simulink model "motorDrivelineElectricalTRQControl"  (R2025b)
settings: Solver=VariableStepAuto  StartTime=0.0  StopTime=0.5  FixedStep=Ts  RelTol=1e-3  AbsTol=1e-3  EnableMultiTasking=on
PreLoadFcn:
  | motorDrivelineElectricalTRQControlParams;
undefined symbols (not defined in the file): elecTRQParams
libraries: nesl_utility x12, fl_lib x10, ee_lib x4, batteryecm_lib x1, eePmsmFieldOrientedControl x1
CloseFcn:
  | try,close(h1_PMSMDrive),end
  | clear h1_PMSMDrive
  | try,close(h2_PMSMDrive),end
  | clear h2_PMSMDrive
  | try,close(h3_PMSMDrive),end
  | clear h3_PMSMDrive
  | try,close(h4_PMSMDrive),end
  | clear h4_PMSMDrive
Description:
  | Three-Phase PMSM Drive
settings Model: Creator=The MathWorks, Inc.  LastModifiedBy=shachind
settings SolverCC: AutoScaleAbsTol=off  MaxConsecutiveMinStep=2  ZeroCrossAlgorithm=Adaptive  AlgebraicLoopSolver=TrustRegion  MaxZcPerStep=1.0
settings DataIOCC: LimitDataPoints=on  MaxDataPoints=690000  SaveFormat=Array  SignalLogging=off
settings OptimizationCC: ReuseModelBlockBuffer=off  LifeSpan=inf
settings DebuggingCC: MaxConsecutiveZCsMsg=none  IgnoredZcDiagnostic=none  UnconnectedInputMsg=warning  UnconnectedOutputMsg=warning  UnconnectedLineMsg=warning  AllowSymbolicDim=off  PregeneratedLibrarySubsystemCodeDiagnostic=none  SFUnexpectedBacktrackingDiag=warning  SFNoUnconditionalDefaultTransitionDiag=warning  SFExecutionAtInitializationDiag=none  ArithmeticOperatorsInVariantConditions=warning
settings HardwareCC: ProdBitPerPointer=32.0  ProdBitPerSizeT=32.0  ProdBitPerPtrDiffT=32.0  ProdLargestAtomicFloat=None  ProdIntDivRoundTo=Undefined  ProdEndianess=Unspecified  ProdWordSize=32.0  ProdHWDeviceType=32-bit Generic
settings ModelReferenceCC: EnableRefExpFcnMdlSchedulingChecks=on  PropagateSignalLabelsOutOfModel=off
settings SFSimCC: SimUseLocalCustomCode=off
settings RTWCC: RTWUseLocalCustomCode=off  GPUComputeCapability=3.5  DLArmComputeVersion=19.05
settings CodeAppCC: StateflowObjectComments=on
settings GRTTargetCC: TargetLangStandard=C89/C90 (ANSI)
settings ConfigComp: CovMetricSettings=dw  CovSaveCumulativeToWorkspaceVar=on  CovSaveSingleToWorkspaceVar=on  CovExternalEMLEnable=off  CovSFcnEnable=off
settings SimscapeCC: SimscapeLogType=all  SimscapeLogName=simlogmotorDrivelineElectricalTRQControl  SimscapeLogLimitData=off  SimscapeLogDataHistory=690000.0

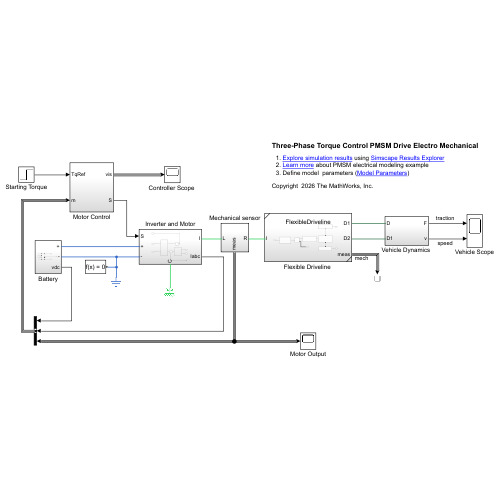
[thumbnail: Simulink's stored preview of the top-level diagram]
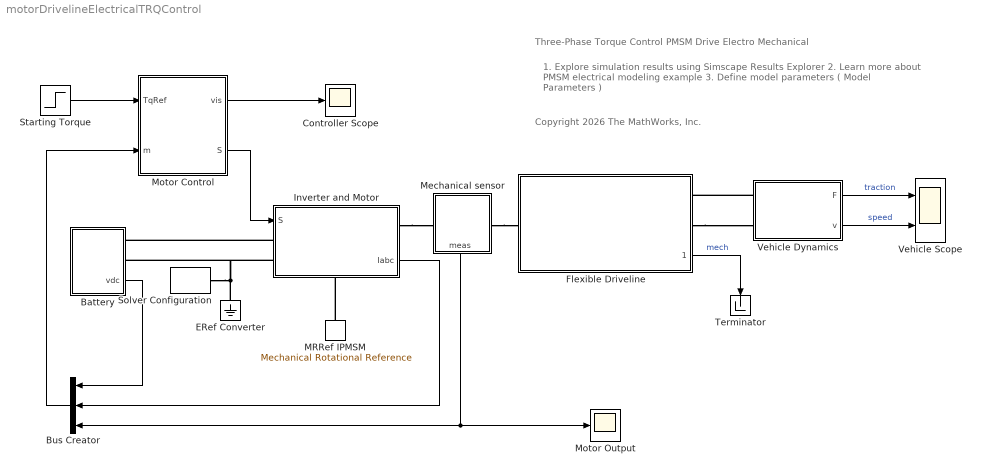
== system motorDrivelineElectricalTRQControl ==
  note: Three-Phase Torque Control PMSM Drive Electro Mechanical
  note: 1. Explore simulation results using Simscape Results Explorer
      | 2. Learn more about PMSM electrical modeling example
      | 3. Define model parameters ( Model Parameters )
  note: Copyright 2026 The MathWorks, Inc.
  Battery : Subsystem
      settings: PortSchema="{\"entries\":[{\"content\":{\"sides\":[{\"content\":{},\"type\":\"ConnectorPlacement.EquallySpacedRectSide\",\"uuid\":\"3e4692f5-9bd7-4a52-b9b4-dbfde3041e1b\"},{\"content\":{\"connectorIds\":[\"RConn1\",\"RConn2\",\"Out1\"],\"side\":\"RIGHT\"},\"type\":\"ConnectorPlacement.EquallySpacedRectSide\",\"uuid\":\"34170655-efd1-4725-b892-0490a88cd6b3\"},{\"content\":{\"side\":\"TOP\"},\"type\":\"ConnectorPlacement.EquallySpacedRectSide\",\"uuid\":\"051e7fe0-e37a-4958-8dcf-c73d0495e662\"},{\"content\":{\"side\":\"BOTTOM\"},\"type\":\"ConnectorPlacement.EquallySpacedRectSide\",\"uuid\":\"b1fc2594-e254-4206-a57f-073d724655f5\"}]},\"type\":\"ConnectorPlacement.EquallySpacedConnector\",\"uuid\":\"32af2e3c-f8f5-43b3-81bc-9b6fee978ebc\"}],\"packageUris\":[\"http://schema.mathworks.com/mf0/Connector/R2020b\"],\"version\":\"1.0\"}"
  Bus Creator : BusCreator  Inputs=3
  "Controller Scope " : Scope
      settings: ActiveDisplayYMinimum=-362.43334059575272  ActiveDisplayYMaximum=223.49886029038308
  ERef Converter : fl_lib/Electrical/Electrical Elements/Electrical Reference
  "Flexible Driveline " : Subsystem  ReferencedSubsystem=FlexibleDriveline
      settings: PortSchema="{\"entries\":[{\"content\":{\"sides\":[{\"content\":{\"connectorIds\":[\"LConn1\"]},\"type\":\"ConnectorPlacement.EquallySpacedRectSide\",\"uuid\":\"b641ef45-b70e-4196-8c46-ca8cab1c313e\"},{\"content\":{\"connectorIds\":[\"RConn1\",\"RConn2\",\"Out1\"],\"side\":\"RIGHT\"},\"type\":\"ConnectorPlacement.EquallySpacedRectSide\",\"uuid\":\"8a51df86-71ec-48ae-9cae-5a3f671581d5\"},{\"content\":{\"side\":\"TOP\"},\"type\":\"ConnectorPlacement.EquallySpacedRectSide\",\"uuid\":\"1e4e883b-852e-4889-9310-df4ba72c2f7b\"}]},\"type\":\"ConnectorPlacement.EquallySpacedConnector\",\"uuid\":\"d094a044-8f93-4a08-a2c2-1a95b6407718\"}],\"packageUris\":[\"http://schema.mathworks.com/mf0/Connector/R2020b\"],\"version\":\"1.0\"}"
  Inverter and Motor : Subsystem
      settings: PortSchema="{\"entries\":[{\"content\":{\"sides\":[{\"content\":{\"connectorIds\":[\"In1\",\"LConn1\",\"LConn2\"]},\"type\":\"ConnectorPlacement.EquallySpacedRectSide\",\"uuid\":\"79886a42-20e0-415e-bc70-e8f3f934141c\"},{\"content\":{\"connectorIds\":[\"RConn1\",\"Out1\"],\"side\":\"RIGHT\"},\"type\":\"ConnectorPlacement.EquallySpacedRectSide\",\"uuid\":\"24b2e8ac-3a57-4634-be65-eb2e006efc4c\"},{\"content\":{\"side\":\"TOP\"},\"type\":\"ConnectorPlacement.EquallySpacedRectSide\",\"uuid\":\"fad38467-7104-4348-9d8d-90e314d27ae8\"},{\"content\":{\"connectorIds\":[\"RConn2\"],\"side\":\"BOTTOM\"},\"type\":\"ConnectorPlacement.EquallySpacedRectSide\",\"uuid\":\"f364d779-702d-4da4-a90d-a3d412e5412e\"}]},\"type\":\"ConnectorPlacement.EquallySpacedConnector\",\"uuid\":\"c4c0e35c-7ac9-412b-ab3f-384c1c56da6e\"}],\"packageUris\":[\"http://schema.mathworks.com/mf0/Connector/R2020b\"],\"version\":\"1.0\"}"
  MRRef IPMSM : fl_lib/Mechanical/Rotational Elements/Mechanical Rotational Reference
  Mechanical sensor : Subsystem
      settings: PortSchema="{\"entries\":[{\"content\":{\"sides\":[{\"content\":{\"connectorIds\":[\"LConn1\"]},\"type\":\"ConnectorPlacement.EquallySpacedRectSide\",\"uuid\":\"9d0b7eaf-5dbc-4711-a9f9-5254d5ad2438\"},{\"content\":{\"connectorIds\":[\"RConn1\"],\"side\":\"RIGHT\"},\"type\":\"ConnectorPlacement.EquallySpacedRectSide\",\"uuid\":\"1084bd7e-accf-404d-815d-6b48331d5fd1\"},{\"content\":{\"side\":\"TOP\"},\"type\":\"ConnectorPlacement.EquallySpacedRectSide\",\"uuid\":\"4e1c109f-5704-45c2-8a88-7bde344122da\"},{\"content\":{\"connectorIds\":[\"Out1\"],\"side\":\"BOTTOM\"},\"type\":\"ConnectorPlacement.EquallySpacedRectSide\",\"uuid\":\"dec56fa8-46a5-4b4d-8685-27108f0f957c\"}]},\"type\":\"ConnectorPlacement.EquallySpacedConnector\",\"uuid\":\"e6b98985-8de9-437e-9e9a-976cda41402d\"}],\"packageUris\":[\"http://schema.mathworks.com/mf0/Connector/R2020b\"],\"version\":\"1.0\"}"
  Motor Control : Subsystem
  Motor Output : Scope
      settings: ActiveDisplayYMinimum=-152.33940612292497  ActiveDisplayYMaximum=237.58310712785936  DataLoggingVariableName=ScopeData2
  Solver Configuration : nesl_utility/Solver Configuration  PhysicalDomain=network_engine_domain  SubClassName=solver  LeftPortType=input  RightPortType=generic  Tones=[]  Harmonics=[]  SimulateNoise=off  Profile=off  UseLocalSampling=off  EnableSwitchedLinearOptims=on  FrequencyDomain=off  UseCCode=off  RelTol=0.001  AbsTol=0.001  MinStep=1e-09  ToWorkspace=off  RevertToSquareIcSolve=off  NumHomotopyIterations=100  PhasorMode=off  PhasorModeNumHarmonics=1  ConsistencySolver=NEWTON_XTOL_AFTER_FTOL  IndexReductionMethod=DerivativeReplacement  DoDC=off  ResidualTolerance=1e-09  ConsistencyTolSource=GLOBAL  ConsistencyAbsTol=0.001  ConsistencyRelTol=0.001  ConsistencyTolFactor=0.001  UseLocalSolver=on  LocalSolverChoice=NE_BACKWARD_EULER_ADVANCER  ResolveIndetEquations=on  FunctionEvalNumThread=1  LocalSolverSampleTime=5e-5  DoFixedCost=off  MaxNonlinIter=3  MaxModeIter=2  ComputeImpulses=off  ImpulseIterations=2  LinearAlgebra=auto  LinearAlgebraNumThread=0  EquationFormulation=NE_TIME_EF  DelaysMemoryBudget=1024  AutomaticFiltering=on  FilteringTimeConstant=0.001  PartitionStorageMethod=AS_NEEDED  PartitionMemoryBudget=1024  PartitionMethod=ROBUST  MultibodyUseLocalSolver=off  MultibodyLocalSolverChoice=ODE1  MultibodyLocalSolverSampleTime=0.001
  Starting Torque : Step  Time=0.01  After=50  SampleTime=0
  Terminator : Terminator
  "Vehicle Dynamics " : Subsystem
  Vehicle Scope : Scope  NumInputPorts=2
      settings: ActiveDisplayYMinimum=-534.32238927144817  ActiveDisplayYMaximum=4808.9015034430349
  wires:
  "Vehicle Dynamics "/1(F) -> Vehicle Scope/1  "traction"
  "Vehicle Dynamics "/2(v) -> Vehicle Scope/2  "speed"
  Bus Creator/1 -> Motor Control/2(m)
  Starting Torque/1 -> Motor Control/1(TqRef)
  Battery/1(vdc) -> Bus Creator/1
  Motor Control/2(S) -> Inverter and Motor/1(S)
  Inverter and Motor/1(Iabc) -> Bus Creator/2
  Mechanical sensor/1(meas) -> Motor Output/1, Bus Creator/3
  "Flexible Driveline "/1 -> Terminator/1  "mech"
  Motor Control/1(vis) -> "Controller Scope "/1
  connections:
  "Vehicle Dynamics "/LConn1 -- "Flexible Driveline "/RConn1
  "Flexible Driveline "/RConn2 -- "Vehicle Dynamics "/LConn2
  Solver Configuration/RConn1 -- ERef Converter/LConn1 -- Inverter and Motor/LConn2 -- Battery/RConn2
  Inverter and Motor/LConn1 -- Battery/RConn1
  MRRef IPMSM/LConn1 -- Inverter and Motor/RConn2
  Inverter and Motor/RConn1 -- Mechanical sensor/RConn1
  Mechanical sensor/LConn1 -- "Flexible Driveline "/LConn1

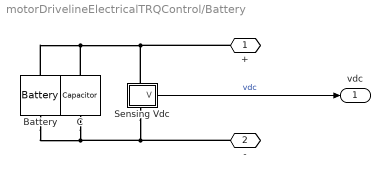
== system motorDrivelineElectricalTRQControl/Battery ==
  Battery : batteryecm_lib/Battery  Vnom=450 V  prm_dir=1  R1_dis=2 Ohm  R1_ch=2 Ohm  R1=0.001 Ohm  prm_AH=1  AH=300 hr*A  V1=V1 V  AH1=100 hr*A  prm_R2=1  R2=2000 Ohm  Tmeas=298.15 K  charge_measurement_port=simscape.enum.battery.enable.no  prm_dyn=1  Rp1=0.005 Ohm  tau1=30 s  Rp2=0.005 Ohm  tau2=30 s  Rp3=0.005 Ohm  tau3=30 s  Rp4=0.005 Ohm  tau4=30 s  Rp5=0.005 Ohm  tau5=30 s  prm_fade=1  N_fade=100  AH_fade=45 hr*A  R1_fade=2.02 Ohm  R1_ch_fade=2.02 Ohm  V1_fade=10.35 V  prm_age=1  prm_age_OCV=1  OCV_age=0.9  SOC_age=60  Tmeas_age=298.15 K  delta_time_age_vec=[0] d  temperature_age_vec=[273] K  OCV_scaling_age=2.2134e6  OCV_offset_age=1.632e6  temp_exp_age=0.515833569 V  t_exp_age=0.75  Vnom_T2=12 V  R1_T2=2.2 Ohm  R1_T2_dis=2.2 Ohm  R1_T2_ch=2.2 Ohm  V1_T2=11.4 V  R2_T2=2200 Ohm  Rp1_T2=0.005 Ohm  tau1_T2=30 s  Rp2_T2=0.005 Ohm  tau2_T2=30 s  Rp3_T2=0.005 Ohm  tau3_T2=30 s  Rp4_T2=0.005 Ohm  tau4_T2=30 s  Rp5_T2=0.005 Ohm  tau5_T2=30 s  Tmeas2=273.15 K  thermal_port=simscape.enum.thermaleffects.omit  thermal_mass=30000 J/K  i_specify=off  i_priority=None  i=0 A  i_nominal_specify=off  i_nominal_value=1  i_nominal_unit=A  v_specify=off  v_priority=None  v=0 V  v_nominal_specify=off  v_nominal_value=1  v_nominal_unit=V  charge_specify=on  charge_priority=High  charge=elecTRQParams.battery.ah0 hr*A  charge_nominal_specify=off  charge_nominal_value=1  charge_nominal_unit=A*hr  num_cycles_specify=off  num_cycles_priority=High  num_cycles=0  num_cycles_nominal_specify=off  num_cycles_nominal_value=1  num_cycles_nominal_unit=1  temperature_specify=off  temperature_priority=High  temperature=298.15 K  temperature_nominal_specify=off  temperature_nominal_value=1  temperature_nominal_unit=K
  C : fl_lib/Electrical/Electrical Elements/Capacitor  c=elecTRQParams.battery.cdc F  r=1e-6 Ohm  g=0 1/Ohm  i_specify=off  i_priority=None  i=0 A  i_nominal_specify=off  i_nominal_value=1  i_nominal_unit=A  v_specify=off  v_priority=None  v=0 V  v_nominal_specify=off  v_nominal_value=1  v_nominal_unit=V  vc_specify=on  vc_priority=None  vc=elecTRQParams.battery.vnom V  vc_nominal_specify=off  vc_nominal_value=1  vc_nominal_unit=V
  Sensing Vdc : Subsystem
      settings: PortSchema="{\"entries\":[{\"content\":{\"sides\":[{\"content\":{\"connectorIds\":[\"LConn1\"]},\"type\":\"ConnectorPlacement.EquallySpacedRectSide\",\"uuid\":\"bc3757cc-4537-444e-89af-7b7d8c8c1fa7\"},{\"content\":{\"connectorIds\":[\"RConn1\"],\"side\":\"RIGHT\"},\"type\":\"ConnectorPlacement.EquallySpacedRectSide\",\"uuid\":\"908bf4c4-26f6-4d8a-bcf8-68236027f5f8\"},{\"content\":{\"side\":\"TOP\"},\"type\":\"ConnectorPlacement.EquallySpacedRectSide\",\"uuid\":\"33f228db-ba47-4718-96dc-a72de309ae8c\"},{\"content\":{\"connectorIds\":[\"Out1\"],\"side\":\"BOTTOM\"},\"type\":\"ConnectorPlacement.EquallySpacedRectSide\",\"uuid\":\"d9b66c7e-0954-4c47-8bcc-77bf13ff573c\"}]},\"type\":\"ConnectorPlacement.EquallySpacedConnector\",\"uuid\":\"345f3578-0572-4e64-b2f3-84728129a12d\"}],\"packageUris\":[\"http://schema.mathworks.com/mf0/Connector/R2020b\"],\"version\":\"1.0\"}"
  + : PMIOPort  Side=Right
  - : PMIOPort  Port=2  Side=Right
  vdc : Outport
  wires:
  Sensing Vdc/1(V) -> vdc/1  "vdc"
  connections:
  C/LConn1 -- +/RConn1 -- Sensing Vdc/LConn1 -- Battery/LConn1
  -/RConn1 -- Battery/RConn1 -- C/RConn1 -- Sensing Vdc/RConn1

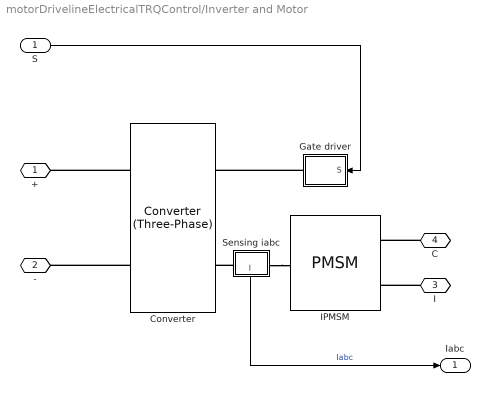
== system motorDrivelineElectricalTRQControl/Inverter and Motor ==
  S : Inport
  Converter : ee_lib/Semiconductors & Converters/Converters/Converter (Three-Phase)  port_option=ee.enum.threePhasePort.composite  fidelity_option=ee.enum.converters.fidelity.detailed  device_type=ee.enum.converters.switchingdevice.ideal  showThermalPort=false  K=0  Vth=0.5 V  Vgt=1 V  Vgt_off=-1 V  Ih=1 A  Vf=0.8 V  Ron=0.001 Ohm  Rds=0.001 Ohm  Goff=1e-5 1/Ohm  Eon_scalar=22.86e-3 J  Eoff_scalar=17.14e-3 J  Eoff_natural_commutation=10e-3 J  Voff=300 V  Iout_scalar=600 A  onCurrentMeasDelay=0 s  useCurrentFromPreviousCycle=false  useVoltageFromPreviousCycle=false  diode_param=ee.enum.converters.protectiondiode.nodynamics  diode_Vf=0.8 V  diode_Ron=0.001 Ohm  diode_Goff=1e-5 1/Ohm  diode_C=50 nF  diode_iRM=-235 A  diode_iF=300 A  diode_idot=-50 A/us  diode_trr_param=1  diode_trr_factor=3  diode_trr=15 us  diode_Qrr=1.5e+3 s*uA  diode_rec_loss_model=ee.enum.diode.reverseRecoveryModel.fixed  diode_ErecVal=0 J  diode_scaleWithIandV=false  diode_ErecMat=zeros(2, 3) J  diode_TjrecVec=[298.15, 398.15] K  diode_IfrecVec=[.1, 1, 10] A  diode_IrecVal=10 A  diode_VrecVal=10 V  diode_tFilter=1 / 1000 / 100 s  thermal_network_parameterization=ee.enum.thermalNetworkTopology.external  Rth=[.08, .5] K/W  Rth_Cauer=[.08, .1, .5] K/W  Rth_Foster=[.08, .14, .22, .16] K/W  thermal_mass_parameterization=ee.enum.thermalNetwork.timeconstant  thermal_mass=[.01, .5] J/K  thermal_mass_Cauer=[.01, .1, .5] J/K  thermal_mass_Foster=[.001, .005, .05, .5] J/K  thermal_time_constant=[.001, .2] s  thermal_time_constant_Cauer=[.001, .1, .2] s  thermal_time_constant_Foster=[7e-05, .0007, .01, .08] s  thermal_mass_initial_temperatures=[25, 25] degC  thermal_mass_initial_temperatures_Cauer=[25, 25, 25] degC  junction_thermal_mass=0.01 J/K  Tvec_initial_Foster=[25, 25, 25, 25] degC  snubber_type=0  Cs=1e-7 F  Rs=0.1 Ohm  Vce_loss=[0, 150, 300] V
  Gate driver : Subsystem
  IPMSM : ee_lib/Electromechanical/Permanent Magnet/PMSM  port_option=ee.enum.threePhasePort.composite  winding_type=ee.enum.statorconnection.wye  machine_param=ee.enum.pmsm.parameterization.constant  nPolePairs=elecTRQParams.motor.p  pmflux_param=ee.enum.pmflux.fluxlinkage  pm_flux_linkage=elecTRQParams.motor.psim Wb  torque_constant=0.18 N*m/A  back_emf_constant=0.18 V/(rad/s)  stator_param=ee.enum.statorparam.LdLqL0  Ld=elecTRQParams.motor.ld H  Lq=elecTRQParams.motor.lq H  idVec=[-200, 0, 200] A  iqVec=[-200, 0, 200] A  LdMatrix=0.0002 * ones(3, 3) H  LqMatrix=0.0002 * ones(3, 3) H  PmMatrix=0.1 * ones(3, 3) Wb  ktMatrix=0.18 * ones(3, 3) N*m/A  keMatrix=0.18 * ones(3, 3) V/(rad/s)  L0=elecTRQParams.motor.l0 H  Ls=0.0002 H  Lm=0.00002 H  Ms=0.00002 H  Rs=elecTRQParams.motor.rs Ohm  zero_sequence=ee.enum.park.zerosequence.exclude  axes_param=ee.enum.rotorangle.qaxis  loss_param=ee.enum.ironloss.none  losses_oc=[0, 0, 0] W  losses_sc=[0, 0, 0] W  f_losses=60 Hz  Isc_losses=95 A  J=0.01 kg*m^2  lam=0.1 N*m/(rad/s)  i_d_specify=off  i_d_priority=None  i_d=0 A  i_d_nominal_specify=off  i_d_nominal_value=1  i_d_nominal_unit=A  i_q_specify=off  i_q_priority=None  i_q=0 A  i_q_nominal_specify=off  i_q_nominal_value=1  i_q_nominal_unit=A  torque_specify=off  torque_priority=None  torque=0 N*m  torque_nominal_specify=off  torque_nominal_value=1  torque_nominal_unit=N*m  angular_velocity_specify=on  angular_velocity_priority=None  angular_velocity=0 rad/s  angular_velocity_nominal_specify=off  angular_velocity_nominal_value=1  angular_velocity_nominal_unit=rpm  angular_position_specify=on  angular_position_priority=High  angular_position=0 rad  angular_position_nominal_specify=off  angular_position_nominal_value=1  angular_position_nominal_unit=deg  alpha=3.93e-3 1/K  alpha_flux=-0.001 1/K  Tmeas=298.15 K  stator_thermal_mass=100 J/K  rotor_thermal_mass=200 J/K  Rm_percent_rotor=90  Rd_percent_rotor=30  temperatureA_specify=off  temperatureA_priority=High  temperatureA=25 degC  temperatureA_nominal_specify=off  temperatureA_nominal_value=1  temperatureA_nominal_unit=degC  temperatureB_specify=off  temperatureB_priority=High  temperatureB=25 degC  temperatureB_nominal_specify=off  temperatureB_nominal_value=1  temperatureB_nominal_unit=degC  temperatureC_specify=off  temperatureC_priority=High  temperatureC=25 degC  temperatureC_nominal_specify=off  temperatureC_nominal_value=1  temperatureC_nominal_unit=degC  temperatureR_specify=off  temperatureR_priority=High  temperatureR=25 degC  temperatureR_nominal_specify=off  temperatureR_nominal_value=1  temperatureR_nominal_unit=degC
      settings: InternalSimscapePortConfiguration="{\"Bottom\":[],\"Left\":[{\"id\":\"N\",\"label\":\"~\",\"type\":\"foundation.electrical.three_phase\"}],\"Right\":[{\"id\":\"R\",\"label\":\"R\",\"type\":\"foundation.mechanical.rotational.rotational\"},{\"id\":\"C\",\"label\":\"C\",\"type\":\"foundation.mechanical.rotational.rotational\"}],\"Top\":[]}"
  Sensing iabc : Subsystem
      settings: PortSchema="{\"entries\":[{\"content\":{\"sides\":[{\"content\":{\"connectorIds\":[\"LConn1\"]},\"type\":\"ConnectorPlacement.EquallySpacedRectSide\",\"uuid\":\"bc3757cc-4537-444e-89af-7b7d8c8c1fa7\"},{\"content\":{\"connectorIds\":[\"RConn1\"],\"side\":\"RIGHT\"},\"type\":\"ConnectorPlacement.EquallySpacedRectSide\",\"uuid\":\"908bf4c4-26f6-4d8a-bcf8-68236027f5f8\"},{\"content\":{\"connectorIds\":[],\"side\":\"TOP\"},\"type\":\"ConnectorPlacement.EquallySpacedRectSide\",\"uuid\":\"33f228db-ba47-4718-96dc-a72de309ae8c\"},{\"content\":{\"connectorIds\":[\"Out1\"],\"side\":\"BOTTOM\"},\"type\":\"ConnectorPlacement.EquallySpacedRectSide\",\"uuid\":\"3b1d40a5-3c80-431c-8111-df754e0c502b\"}]},\"type\":\"ConnectorPlacement.EquallySpacedConnector\",\"uuid\":\"345f3578-0572-4e64-b2f3-84728129a12d\"}],\"packageUris\":[\"http://schema.mathworks.com/mf0/Connector/R2020b\"],\"version\":\"1.0\"}"
  + : PMIOPort  Side=Left
  - : PMIOPort  Port=2  Side=Left
  I : PMIOPort  Port=3  Side=Right
  C : PMIOPort  Port=4  Side=Right
  Iabc : Outport
  wires:
  Sensing iabc/1(I) -> Iabc/1  "Iabc"
  S/1 -> Gate driver/1(S)
  connections:
  Sensing iabc/RConn1 -- IPMSM/LConn1
  C/RConn1 -- IPMSM/RConn2
  Converter/RConn2 -- -/RConn1
  Sensing iabc/LConn1 -- Converter/LConn2
  Gate driver/RConn1 -- Converter/LConn1
  Converter/RConn1 -- +/RConn1
  I/RConn1 -- IPMSM/RConn1

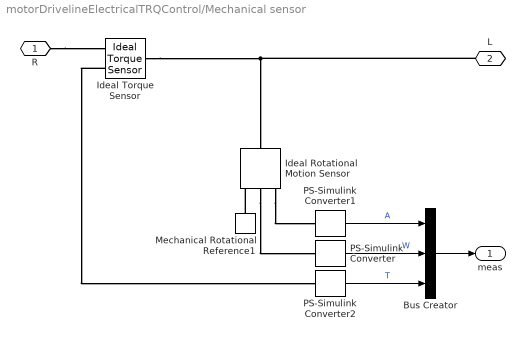
== system motorDrivelineElectricalTRQControl/Mechanical sensor ==
  Bus Creator : BusCreator  Inputs=3
  Ideal Rotational Motion Sensor : fl_lib/Mechanical/Mechanical Sensors/Ideal Rotational Motion Sensor  reference=foundation.enum.MeasurementReference.difference  acceleration_port=false  velocity_port=true  position_port=true  wrap_angle=simscape.enum.onoff.off  offset=0 deg
  Ideal Torque Sensor : fl_lib/Mechanical/Mechanical Sensors/Ideal Torque Sensor
  Mechanical Rotational Reference1 : fl_lib/Mechanical/Rotational Elements/Mechanical Rotational Reference
  PS-Simulink Converter : nesl_utility/PS-Simulink Converter  PhysicalDomain=network_engine_domain  SubClassName=ps_output  LeftPortType=input  RightPortType=output  PseudoPeriodic=off  Frequencies=[]  VectorFormat=1-D array  Unit=rad/s  AffineConversion=off
  PS-Simulink Converter1 : nesl_utility/PS-Simulink Converter  PhysicalDomain=network_engine_domain  SubClassName=ps_output  LeftPortType=input  RightPortType=output  PseudoPeriodic=off  Frequencies=[]  VectorFormat=1-D array  Unit=rad  AffineConversion=off
  PS-Simulink Converter2 : nesl_utility/PS-Simulink Converter  PhysicalDomain=network_engine_domain  SubClassName=ps_output  LeftPortType=input  RightPortType=output  PseudoPeriodic=off  Frequencies=[]  VectorFormat=1-D array  Unit=N*m  AffineConversion=off
  R : PMIOPort  Side=Left
  L : PMIOPort  Port=2  Side=Right
  meas : Outport  VectorParamsAs1DForOutWhenUnconnected=off
  wires:
  Bus Creator/1 -> meas/1
  PS-Simulink Converter1/1 -> Bus Creator/1  "A"
  PS-Simulink Converter/1 -> Bus Creator/2  "W"
  PS-Simulink Converter2/1 -> Bus Creator/3  "T"
  connections:
  L/RConn1 -- Ideal Torque Sensor/LConn1 -- Ideal Rotational Motion Sensor/LConn1
  Ideal Rotational Motion Sensor/RConn2 -- PS-Simulink Converter/LConn1
  Ideal Rotational Motion Sensor/RConn3 -- PS-Simulink Converter1/LConn1
  Mechanical Rotational Reference1/LConn1 -- Ideal Rotational Motion Sensor/RConn1
  Ideal Torque Sensor/RConn2 -- PS-Simulink Converter2/LConn1
  R/RConn1 -- Ideal Torque Sensor/RConn1

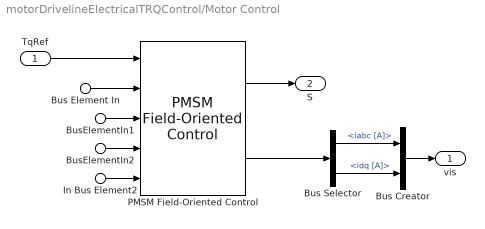
== system motorDrivelineElectricalTRQControl/Motor Control ==
  TqRef : Inport
  Bus Element In : Inport  Port=2  PortName=m  Element=Iabc
  In Bus Element2 : Inport  Port=2  PortName=m  Element=vdc
  BusElementIn1 : Inport  Port=2  PortName=m  Element=signal3.W
  BusElementIn2 : Inport  Port=2  PortName=m  Element=signal3.A
  Bus Creator : BusCreator  Inputs=2
  Bus Selector : BusSelector  OutputSignals=iabc [A],idq [A]
  PMSM Field-Oriented Control : eePmsmFieldOrientedControl/PMSM Field-Oriented Control  winding_type=Wye-wound  CtrlMode=Torque control  Vnom=elecTRQParams.battery.vnom  Pmax=28902.6524  Tmax=elecTRQParams.motor.tmax  p=elecTRQParams.motor.p  Vdc_on=100  Ts=elecTRQParams.control.ts  Tsc=elecTRQParams.control.tsc  CtrlType=PI control  Kp_w=1  Ki_w=1  Kv_w=1  Kaw_w=1  RefType=Zero d-axis control  rpmVec=[0, 3000]  TqVec=[-100, 0, 100]  VdcVec=[300, 350]  PWMMode=SVM: space vector modulation  ModFactor=1  idMatrix=zeros(2,3,2)  iqMatrix=zeros(2,3,2)  psim=elecTRQParams.motor.psim  Ld=0.00024  Lq=0.00029  Rs=0.01  AxisAlignment=Q-axis  Kp_id=elecTRQParams.piId.kp  Ki_id=elecTRQParams.piId.ki  Kaw_id=1  Kp_iq=elecTRQParams.piIq.kp  Ki_iq=elecTRQParams.piIq.ki  Kaw_iq=1  AxisPrio=Q-axis  ActZC=off  ActFF=on  ParamTypeFF=Constant parameters  LdFF=elecTRQParams.motor.ld  LqFF=elecTRQParams.motor.lq  psimFF=elecTRQParams.motor.psim  idVect=[-200, 0, 200]  iqVect=[-200, 0, 200]  LdMatrix=0.0002 * ones(3, 3)  LqMatrix=0.0002 * ones(3, 3)  psimMatrix=0.04 * ones(3, 3)  CPWMMode=SVM: space vector modulation  fsw=elecTRQParams.control.fsw
      settings: LibrarySourceBlock=|
      | ee_sl_lib/PMSM Control/PMSM Field-Oriented
      | Control
  vis : Outport
  S : Outport  Port=2
  wires:
  PMSM Field-Oriented Control/1 -> S/1
  TqRef/1 -> PMSM Field-Oriented Control/1
  Bus Element In/1 -> PMSM Field-Oriented Control/2
  In Bus Element2/1 -> PMSM Field-Oriented Control/5
  BusElementIn1/1 -> PMSM Field-Oriented Control/3
  BusElementIn2/1 -> PMSM Field-Oriented Control/4
  PMSM Field-Oriented Control/2 -> Bus Selector/1
  Bus Selector/1 -> Bus Creator/1  "<iabc [A]>"
  Bus Creator/1 -> vis/1
  Bus Selector/2 -> Bus Creator/2  "<idq [A]>"

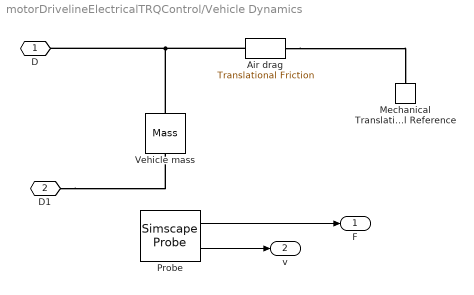
== system motorDrivelineElectricalTRQControl/Vehicle Dynamics  ==
  "Air drag " : fl_lib/Mechanical/Translational Elements/Translational Friction  brkwy_frc=300 N  brkwy_vel=0.01 m/s  Col_frc=150 N  visc_coef=7.25 N*s/m  v_specify=off  v_priority=None  v=0 m/s  v_nominal_specify=off  v_nominal_value=1  v_nominal_unit=m/s  f_specify=off  f_priority=None  f=0 N  f_nominal_specify=off  f_nominal_value=1  f_nominal_unit=N
      settings: InternalSimscapePortConfiguration="{\"Bottom\":[],\"Left\":[{\"id\":\"R\",\"label\":\"R\",\"type\":\"foundation.mechanical.translational.translational\"}],\"Right\":[{\"id\":\"C\",\"label\":\"C\",\"type\":\"foundation.mechanical.translational.translational\"}],\"Top\":[]}"
  Mechanical Translational Reference : fl_lib/Mechanical/Translational Elements/Mechanical Translational Reference
  Probe : SimscapeProbe  BoundBlock=581  Variables="{\"f\":{\"Probing\":\"ON\"},\"v\":{\"Probing\":\"ON\"}}"
  Vehicle mass : fl_lib/Mechanical/Translational Elements/Mass  mass=600 kg  num_ports=foundation.enum.numPorts2.two  v_specify=off  v_priority=High  v=0 m/s  v_nominal_specify=off  v_nominal_value=1  v_nominal_unit=m/s  f_specify=off  f_priority=None  f=0 N  f_nominal_specify=off  f_nominal_value=1  f_nominal_unit=N
      settings: InternalSimscapePortConfiguration="{\"Bottom\":[],\"Left\":[{\"id\":\"M\",\"label\":\"\",\"type\":\"foundation.mechanical.translational.translational\"}],\"Right\":[{\"id\":\"N\",\"label\":\"\",\"type\":\"foundation.mechanical.translational.translational\"}],\"Top\":[]}"
  D : PMIOPort  Side=Left
  D1 : PMIOPort  Port=2  Side=Left
  F : Outport
  v : Outport  Port=2
  wires:
  Probe/1 -> F/1
  Probe/2 -> v/1
  connections:
  "Air drag "/RConn1 -- Mechanical Translational Reference/LConn1
  "Air drag "/LConn1 -- Vehicle mass/LConn1 -- D/RConn1
  D1/RConn1 -- Vehicle mass/RConn1

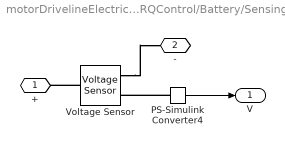
== system motorDrivelineElectricalTRQControl/Battery/Sensing Vdc ==
  PS-Simulink Converter4 : nesl_utility/PS-Simulink Converter  PhysicalDomain=network_engine_domain  SubClassName=ps_output  LeftPortType=input  RightPortType=output  PseudoPeriodic=off  Frequencies=[]  VectorFormat=1-D array  Unit=V  AffineConversion=off
  Voltage Sensor : fl_lib/Electrical/Electrical Sensors/Voltage Sensor
  + : PMIOPort  Side=Left
  - : PMIOPort  Port=2  Side=Right
  V : Outport
  wires:
  PS-Simulink Converter4/1 -> V/1
  connections:
  Voltage Sensor/LConn1 -- +/RConn1
  Voltage Sensor/RConn2 -- -/RConn1
  PS-Simulink Converter4/LConn1 -- Voltage Sensor/RConn1

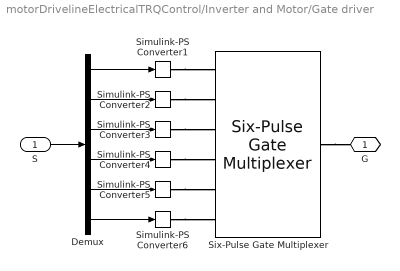
== system motorDrivelineElectricalTRQControl/Inverter and Motor/Gate driver ==
  S : Inport
  Demux : Demux  Outputs=6
  Simulink-PS Converter{1..6} (6 alike) : nesl_utility/Simulink-PS Converter  PhysicalDomain=network_engine_domain  SubClassName=ps_input  LeftPortType=input  RightPortType=output  PseudoPeriodic=off  Frequencies=[]  NoiseDistribution=none  NoiseParameters=[]  Unit=1  AffineConversion=off  FilteringAndDerivatives=zero  SimscapeFilterOrder=1  InputFilterTimeConstant=0.001  UdotUserProvided=1
  Six-Pulse Gate Multiplexer : ee_lib/Semiconductors & Converters/Converters/Six-Pulse Gate Multiplexer  port_option=ee.enum.controlport.ps
  G : PMIOPort  Side=Right
  wires:
  Demux/1 -> Simulink-PS Converter1/1
  S/1 -> Demux/1
  Demux/5 -> Simulink-PS Converter5/1
  Demux/6 -> Simulink-PS Converter6/1
  Demux/4 -> Simulink-PS Converter4/1
  Demux/3 -> Simulink-PS Converter3/1
  Demux/2 -> Simulink-PS Converter2/1
  connections:
  Six-Pulse Gate Multiplexer/RConn1 -- G/RConn1
  Simulink-PS Converter1/RConn1 -- Six-Pulse Gate Multiplexer/LConn1
  Simulink-PS Converter5/RConn1 -- Six-Pulse Gate Multiplexer/LConn5
  Simulink-PS Converter6/RConn1 -- Six-Pulse Gate Multiplexer/LConn6
  Simulink-PS Converter2/RConn1 -- Six-Pulse Gate Multiplexer/LConn2
  Simulink-PS Converter3/RConn1 -- Six-Pulse Gate Multiplexer/LConn3
  Simulink-PS Converter4/RConn1 -- Six-Pulse Gate Multiplexer/LConn4

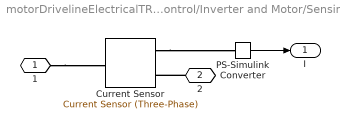
== system motorDrivelineElectricalTRQControl/Inverter and Motor/Sensing iabc ==
  Current Sensor : ee_lib/Sensors & Transducers/Current Sensor (Three-Phase)
  PS-Simulink Converter : nesl_utility/PS-Simulink Converter  PhysicalDomain=network_engine_domain  SubClassName=ps_output  LeftPortType=input  RightPortType=output  PseudoPeriodic=off  Frequencies=[]  VectorFormat=1-D array  Unit=A  AffineConversion=off
  1 : PMIOPort  Side=Left
  2 : PMIOPort  Port=2  Side=Right
  I : Outport
  wires:
  PS-Simulink Converter/1 -> I/1
  connections:
  1/RConn1 -- Current Sensor/LConn1
  2/RConn1 -- Current Sensor/RConn2
  Current Sensor/RConn1 -- PS-Simulink Converter/LConn1
